simulink model "UAV3_GroundStation_05"  (R2026b)
settings: Solver=FixedStepDiscrete  FixedStep=0.1
settings Model: Creator=Ivan  LastModifiedBy=Ivan

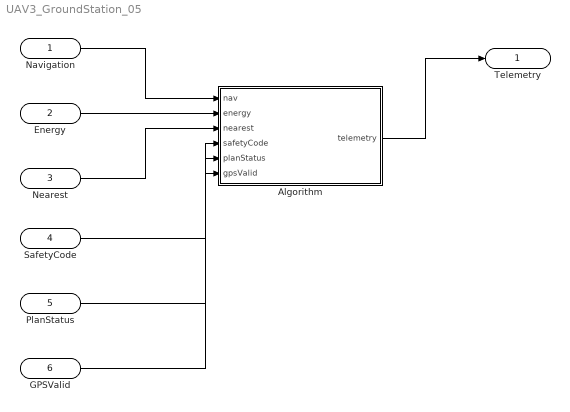
== system UAV3_GroundStation_05 ==
  Navigation : Inport  OutDataTypeStr=double  PortDimensions=[4 1]
  Energy : Inport  Port=2  OutDataTypeStr=double  PortDimensions=[3 1]
  Nearest : Inport  Port=3  OutDataTypeStr=double  PortDimensions=[4 1]
  SafetyCode : Inport  Port=4  OutDataTypeStr=double  PortDimensions=1
  PlanStatus : Inport  Port=5  OutDataTypeStr=double  PortDimensions=[3 1]
  GPSValid : Inport  Port=6  OutDataTypeStr=double  PortDimensions=1
  Algorithm : MATLAB Function  TreatAsAtomicUnit=on
  Telemetry : Outport
  wires:
  Navigation/1 -> Algorithm/1(nav)
  Energy/1 -> Algorithm/2(energy)
  Nearest/1 -> Algorithm/3(nearest)
  SafetyCode/1 -> Algorithm/4(safetyCode)
  PlanStatus/1 -> Algorithm/5(planStatus)
  GPSValid/1 -> Algorithm/6(gpsValid)
  Algorithm/1(telemetry) -> Telemetry/1

== matlab function UAV3_GroundStation_05/Algorithm ==
  data: nav input; telemetry output; energy input; nearest input; safetyCode input; planStatus input; gpsValid input
function telemetry = v3_ground(nav,energy,nearest,safetyCode,planStatus,gpsValid)
%V3_GROUND Fixed-size 9-value ground-station status frame.
% [x;y;speed;battery;nearestDistance;safetyCode;newReplan;
%  knownObstacleCount;gpsAvailable].
%#codegen
telemetry=zeros(9,1);
telemetry(1:2)=nav(1:2);
telemetry(3)=sqrt(sum(nav(3:4).^2));
telemetry(4)=energy(2);
telemetry(5)=nearest(1);
telemetry(6)=safetyCode;
telemetry(7)=planStatus(1);
telemetry(8)=planStatus(2);
telemetry(9)=gpsValid;
end
